simulink library "unit_conversions_lib"  (R2018b)
settings: Solver=VariableStepAuto  StartTime=0.0  StopTime=10.0  RelTol=1e-3
settings Model: Creator=Ybeyer  LastModifiedBy=yannic
settings SFSimCC: SimUseLocalCustomCode=off
settings RTWCC: RTWUseLocalCustomCode=off
settings CodeAppCC: StateflowObjectComments=on

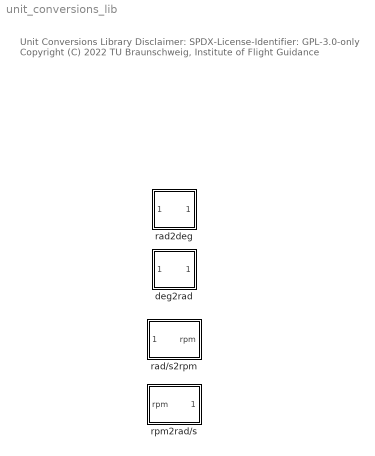
== system unit_conversions_lib ==
  note: Unit Conversions Library
      |
      | Disclaimer:
      | SPDX-License-Identifier: GPL-3.0-only
      |
      | Copyright (C) 2022 TU Braunschweig, Institute of Flight Guidance
  deg2rad : Subsystem
      mask DialogControl DescGroupVar Prompt: deg2rad
      mask DialogControl DescTextVar Prompt: unit conversion from degree to radian
  rad/s2rpm : Subsystem
      mask DialogControl DescGroupVar Prompt: rad/s2rpm
      mask DialogControl DescTextVar Prompt: unit conversion from rad/s to rpm
  rad2deg : Subsystem
      mask DialogControl DescGroupVar Prompt: rad2deg
      mask DialogControl DescTextVar Prompt: unit conversion of radians to degree
  rpm2rad/s : Subsystem
      mask DialogControl DescGroupVar Prompt: rpm2rad/s
      mask DialogControl DescTextVar Prompt: unit conversion from rpm to rad/s

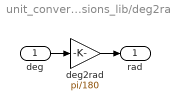
== system unit_conversions_lib/deg2rad ==
  deg : Inport
  deg2rad : Gain  Gain=pi/180
  rad : Outport
  wires:
  deg2rad/1 -> rad/1
  deg/1 -> deg2rad/1

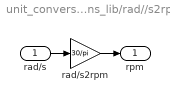
== system unit_conversions_lib/rad//s2rpm ==
  rad/s : Inport
  rad/s2rpm : Gain  Gain=30/pi
  rpm : Outport
  wires:
  rad/s2rpm/1 -> rpm/1
  rad/s/1 -> rad/s2rpm/1

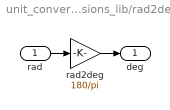
== system unit_conversions_lib/rad2deg ==
  rad : Inport
  rad2deg : Gain  Gain=180/pi
  deg : Outport
  wires:
  rad/1 -> rad2deg/1
  rad2deg/1 -> deg/1

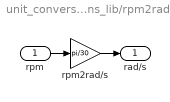
== system unit_conversions_lib/rpm2rad//s ==
  rpm : Inport
  rpm2rad/s : Gain  Gain=pi/30
  rad/s : Outport
  wires:
  rpm2rad/s/1 -> rad/s/1
  rpm/1 -> rpm2rad/s/1
